simulink model "model_23b"  (R2023b)
settings: Solver=ode45  StartTime=TSPAN(1)  StopTime=TSPAN(2)  MaxStep=MaxStep  RelTol=RelTol  AbsTol=AbsTol
values from neighbouring files (symbols this model uses):
  dim_xp = numel(xp_0)    [init.m]
  JSPAN = [0 30*TSPAN(2)]    [init.m]
  parameters = struct()    [init.m]
  TSPAN = [0 600]    [init.m]
  xc_0 = [chi_0;theta_0]    [init.m]
  xp_0 = [p_0;q_0;v_0;o_0]    [init.m]
libraries: HyEQ_Library x2
settings Model: Creator=score  LastModifiedBy=zxz
settings DataIOCC: SaveFormat=Array  ReturnWorkspaceOutputs=off

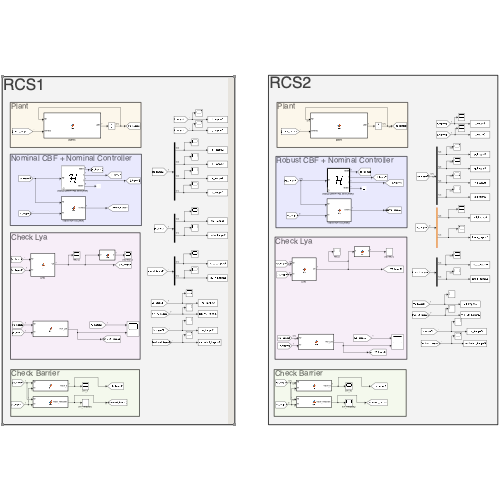
[thumbnail: Simulink's stored preview of the top-level diagram]
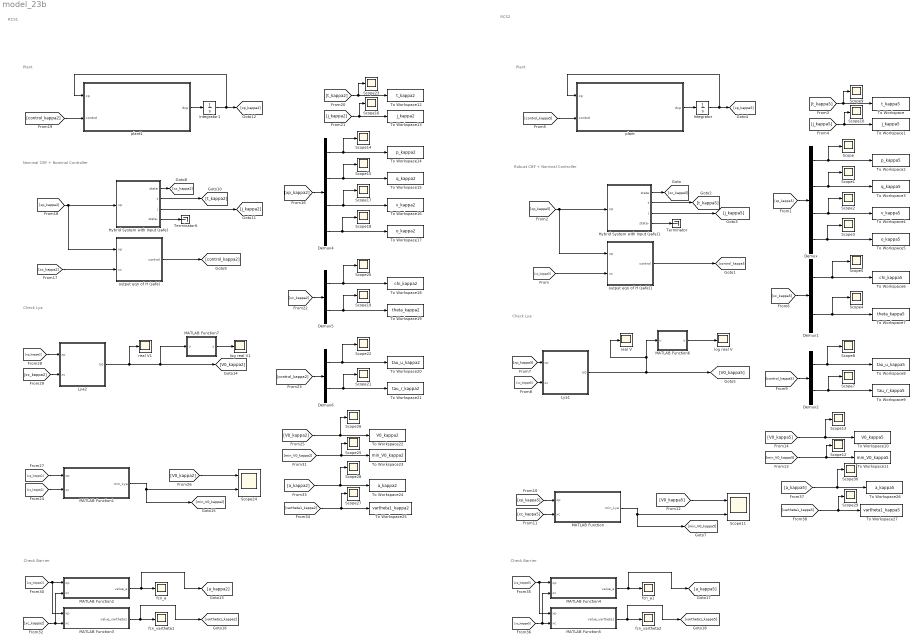
== system model_23b ==
  note: RCS2
  note: RCS1
  note: Check Barrier
  note: Check Lya
  note: Plant
  note: Robust CBF + Nominal Controller
  note: Plant
  note: Nominal CBF + Nominal Controller
  note: Check Lya
  note: Check Barrier
  Demux : Demux  Outputs=[2;2;2;1]
  Demux1 : Demux  Outputs=[2;1]
  Demux2 : Demux  Outputs=[1;1]
  Demux4 : Demux  Outputs=[2;2;2;1]
  Demux5 : Demux  Outputs=[2;1]
  Demux6 : Demux  Outputs=[1;1]
  Hybrid System with Input (safe) : Subsystem  LoadFcn=set_param(gcb,'LinkStatus','none')  mask(Hybrid System with Inputs){x0=xc_0, input_dim=dim_xp, parameters=parameters, T=TSPAN(2), J=JSPAN(2), rule=Flow}
      mask prompts: x0 "Initial Condition (column vector)"; input_dim "Input Dimension (positive integer)"; T "Flow Horizon (nonnegative real)"; J "Jump Horizon (nonnegative integer)"; rule "Flow/Jump Priorty Rule"
      mask help:
      | To modify (f, g, C, D) for this block, "Look inside" the block mask by either clicking the down arrow in the lower-left corner or selecting "Mask" > "Look Under Mask" from the context menu.
      |
      | For instructions how to use this block, see the
      mask init:
      | state_dim = numel(x0);
      settings: CopyFcn=|
      | set_param(gcb,'LinkStatus','none'),
      | set_param(gcs, 'MaxStep', 'MaxStep', 'RelTol', 'RelTol','StopTime', 'T')
      mask Help:
      | To modify (f, g, C, D) for this block, "Look inside" the block mask by either clicking the down arrow in the lower-left corner or selecting "Mask" > "Look Under Mask" from the context menu.
      | 
      | The value given in the 'parameters' field is passed as the last input argument for f, g, C, and D. Any MATLAB object can be used, but we recommend using a struct. For example, in the initialization script, a parameters struct can be defined as followed.
      |   parameters = struct();
      |   parameters.A = eye(2);
      |   parameters.B = [1; 0];
      | 
      | The output "x-" is the state output delayed by one integration step. Use this output to break algebraic loops.
      mask TypeOptions x0: Integrator System/x0
      mask TypeOptions T: Integrator System/T
      mask TypeOptions J: Integrator System/J
      mask TypeOptions rule: Jump | Flow | Random
      mask DialogControl Control2 Prompt: Introduction to the HyEQ Simulink-based Library
      mask DialogControl Control2 Callback: hybrid.internal.openHelp('Help_SimulinkLibrary')
      mask DialogControl Container3 Prompt: System Configuration
      mask DialogControl Container2 Prompt: Solver Options
      mask Display:
      | image('Hcal.jpg')
      | port_label('output', 1, 'state')
      | port_label('output', 2, 't')
      | port_label('output', 3, 'j')
      | port_label('output', 4, 'state^-','texmode', 'on')
      | port_label('input', 1, 'xp')
  Hybrid System with Input (safe)1 : Subsystem  LoadFcn=set_param(gcb,'LinkStatus','none')  mask(Hybrid System with Inputs){x0=xc_0, input_dim=dim_xp, parameters=parameters, T=TSPAN(2), J=JSPAN(2), rule=Flow}
      mask prompts: x0 "Initial Condition (column vector)"; input_dim "Input Dimension (positive integer)"; T "Flow Horizon (nonnegative real)"; J "Jump Horizon (nonnegative integer)"; rule "Flow/Jump Priorty Rule"
      mask help:
      | To modify (f, g, C, D) for this block, "Look inside" the block mask by either clicking the down arrow in the lower-left corner or selecting "Mask" > "Look Under Mask" from the context menu.
      |
      | For instructions how to use this block, see the
      mask init:
      | state_dim = numel(x0);
      settings: CopyFcn=|
      | set_param(gcb,'LinkStatus','none'),
      | set_param(gcs, 'MaxStep', 'MaxStep', 'RelTol', 'RelTol','StopTime', 'T')
      mask Help:
      | To modify (f, g, C, D) for this block, "Look inside" the block mask by either clicking the down arrow in the lower-left corner or selecting "Mask" > "Look Under Mask" from the context menu.
      | 
      | The value given in the 'parameters' field is passed as the last input argument for f, g, C, and D. Any MATLAB object can be used, but we recommend using a struct. For example, in the initialization script, a parameters struct can be defined as followed.
      |   parameters = struct();
      |   parameters.A = eye(2);
      |   parameters.B = [1; 0];
      | 
      | The output "x-" is the state output delayed by one integration step. Use this output to break algebraic loops.
      mask TypeOptions x0: Integrator System/x0
      mask TypeOptions T: Integrator System/T
      mask TypeOptions J: Integrator System/J
      mask TypeOptions rule: Jump | Flow | Random
      mask DialogControl Control2 Prompt: Introduction to the HyEQ Simulink-based Library
      mask DialogControl Control2 Callback: hybrid.internal.openHelp('Help_SimulinkLibrary')
      mask DialogControl Container3 Prompt: System Configuration
      mask DialogControl Container2 Prompt: Solver Options
      mask Display:
      | image('Hcal.jpg')
      | port_label('output', 1, 'state')
      | port_label('output', 2, 't')
      | port_label('output', 3, 'j')
      | port_label('output', 4, 'state^-','texmode', 'on')
      | port_label('input', 1, 'xp')
  Integrator : Integrator  InitialCondition=xp_0
  Integrator1 : Integrator  InitialCondition=xp_0
  Lya1 : MATLAB Function  TreatAsAtomicUnit=on
  Lya2 : MATLAB Function  TreatAsAtomicUnit=on
  MATLAB Function : MATLAB Function  TreatAsAtomicUnit=on
  MATLAB Function1 : MATLAB Function  TreatAsAtomicUnit=on
  MATLAB Function2 : MATLAB Function  TreatAsAtomicUnit=on
  MATLAB Function3 : MATLAB Function  TreatAsAtomicUnit=on
  MATLAB Function4 : MATLAB Function  TreatAsAtomicUnit=on
  MATLAB Function5 : MATLAB Function  TreatAsAtomicUnit=on
  MATLAB Function6 : MATLAB Function  TreatAsAtomicUnit=on
  MATLAB Function7 : MATLAB Function  TreatAsAtomicUnit=on
  Scope{,1..5,7..10,12..23,25..30} (28 alike) : Scope
  Scope11 : Scope  NumInputPorts=2
  Scope24 : Scope  NumInputPorts=2
  Terminator : Terminator
  Terminator6 : Terminator
  To Workspace : ToWorkspace  VariableName=t_kappa5  SaveFormat=Structure  SampleTime=-1
      settings: Save2DSignal=2-D array (concatenate along first dimension)
  To Workspace1 : ToWorkspace  VariableName=j_kappa5  SaveFormat=Structure  SampleTime=-1
      settings: Save2DSignal=2-D array (concatenate along first dimension)
  To Workspace10 : ToWorkspace  VariableName=V0_kappa5  SaveFormat=Structure  SampleTime=-1
      settings: Save2DSignal=2-D array (concatenate along first dimension)
  To Workspace11 : ToWorkspace  VariableName=min_V0_kappa5  SaveFormat=Structure  SampleTime=-1
      settings: Save2DSignal=2-D array (concatenate along first dimension)
  To Workspace12 : ToWorkspace  VariableName=t_kappa2  SaveFormat=Structure  SampleTime=-1
      settings: Save2DSignal=2-D array (concatenate along first dimension)
  To Workspace13 : ToWorkspace  VariableName=j_kappa2  SaveFormat=Structure  SampleTime=-1
      settings: Save2DSignal=2-D array (concatenate along first dimension)
  To Workspace14 : ToWorkspace  VariableName=p_kappa2  SaveFormat=Structure  SampleTime=-1
      settings: Save2DSignal=2-D array (concatenate along first dimension)
  To Workspace15 : ToWorkspace  VariableName=q_kappa2  SaveFormat=Structure  SampleTime=-1
      settings: Save2DSignal=2-D array (concatenate along first dimension)
  To Workspace16 : ToWorkspace  VariableName=v_kappa2  SaveFormat=Structure  SampleTime=-1
      settings: Save2DSignal=2-D array (concatenate along first dimension)
  To Workspace17 : ToWorkspace  VariableName=o_kappa2  SaveFormat=Structure  SampleTime=-1
      settings: Save2DSignal=2-D array (concatenate along first dimension)
  To Workspace18 : ToWorkspace  VariableName=chi_kappa2  SaveFormat=Structure  SampleTime=-1
      settings: Save2DSignal=2-D array (concatenate along first dimension)
  To Workspace19 : ToWorkspace  VariableName=theta_kappa2  SaveFormat=Structure  SampleTime=-1
      settings: Save2DSignal=2-D array (concatenate along first dimension)
  To Workspace2 : ToWorkspace  VariableName=p_kappa5  SaveFormat=Structure  SampleTime=-1
      settings: Save2DSignal=2-D array (concatenate along first dimension)
  To Workspace20 : ToWorkspace  VariableName=tau_u_kappa2  SaveFormat=Structure  SampleTime=-1
      settings: Save2DSignal=2-D array (concatenate along first dimension)
  To Workspace21 : ToWorkspace  VariableName=tau_r_kappa2  SaveFormat=Structure  SampleTime=-1
      settings: Save2DSignal=2-D array (concatenate along first dimension)
  To Workspace22 : ToWorkspace  VariableName=V0_kappa2  SaveFormat=Structure  SampleTime=-1
      settings: Save2DSignal=2-D array (concatenate along first dimension)
  To Workspace23 : ToWorkspace  VariableName=min_V0_kappa2  SaveFormat=Structure  SampleTime=-1
      settings: Save2DSignal=2-D array (concatenate along first dimension)
  To Workspace24 : ToWorkspace  VariableName=a_kappa2  SaveFormat=Structure  SampleTime=-1
      settings: Save2DSignal=2-D array (concatenate along first dimension)
  To Workspace25 : ToWorkspace  VariableName=vartheta1_kappa2  SaveFormat=Structure  SampleTime=-1
      settings: Save2DSignal=2-D array (concatenate along first dimension)
  To Workspace26 : ToWorkspace  VariableName=a_kappa5  SaveFormat=Structure  SampleTime=-1
      settings: Save2DSignal=2-D array (concatenate along first dimension)
  To Workspace27 : ToWorkspace  VariableName=vartheta1_kappa5  SaveFormat=Structure  SampleTime=-1
      settings: Save2DSignal=2-D array (concatenate along first dimension)
  To Workspace3 : ToWorkspace  VariableName=q_kappa5  SaveFormat=Structure  SampleTime=-1
      settings: Save2DSignal=2-D array (concatenate along first dimension)
  To Workspace4 : ToWorkspace  VariableName=v_kappa5  SaveFormat=Structure  SampleTime=-1
      settings: Save2DSignal=2-D array (concatenate along first dimension)
  To Workspace5 : ToWorkspace  VariableName=o_kappa5  SaveFormat=Structure  SampleTime=-1
      settings: Save2DSignal=2-D array (concatenate along first dimension)
  To Workspace6 : ToWorkspace  VariableName=chi_kappa5  SaveFormat=Structure  SampleTime=-1
      settings: Save2DSignal=2-D array (concatenate along first dimension)
  To Workspace7 : ToWorkspace  VariableName=theta_kappa5  SaveFormat=Structure  SampleTime=-1
      settings: Save2DSignal=2-D array (concatenate along first dimension)
  To Workspace8 : ToWorkspace  VariableName=tau_u_kappa5  SaveFormat=Structure  SampleTime=-1
      settings: Save2DSignal=2-D array (concatenate along first dimension)
  To Workspace9 : ToWorkspace  VariableName=tau_r_kappa5  SaveFormat=Structure  SampleTime=-1
      settings: Save2DSignal=2-D array (concatenate along first dimension)
  fcn_a : Scope
  fcn_a1 : Scope
  fcn_vartheta1 : Scope
  fcn_vartheta2 : Scope
  log real V : Scope
  log real V1 : Scope
  output eqn of H (safe) : MATLAB Function  TreatAsAtomicUnit=on
  output eqn of H (safe)1 : MATLAB Function  TreatAsAtomicUnit=on
  plant : MATLAB Function  TreatAsAtomicUnit=on
  plant1 : MATLAB Function  TreatAsAtomicUnit=on
  real V : Scope
  real V1 : Scope
  wires:
  Hybrid System with Input (safe)1/4(state-) -> Terminator/1
  Hybrid System with Input (safe)1/2(t) -> [t_kappa5]
  Hybrid System with Input (safe)1/3(j) -> [j_kappa5]
  Hybrid System with Input (safe)1/1(state) -> [xc_kappa5]
  [xp_kappa5] -> output eqn of H (safe)1/1(xp), Hybrid System with Input (safe)1/1(xp)
  [xc_kappa5] -> output eqn of H (safe)1/2(xc)
  output eqn of H (safe)1/1(control) -> [control_kappa5]
  [t_kappa5] -> Scope9/1, To Workspace/1
  [j_kappa5] -> Scope10/1, To Workspace1/1
  plant/1(dxp) -> Integrator/1
  [control_kappa5] -> plant/2(control)
  Integrator/1 -> plant/1(xp), [xp_kappa5]
  [xp_kappa5] -> Demux/1
  [xc_kappa5] -> Demux1/1
  Demux/1 -> Scope/1, To Workspace2/1
  Demux/2 -> Scope1/1, To Workspace3/1
  Demux/3 -> Scope2/1, To Workspace4/1
  Demux/4 -> Scope3/1, To Workspace5/1
  Demux1/2 -> To Workspace7/1, Scope4/1
  Demux1/1 -> Scope5/1, To Workspace6/1
  [xp_kappa5] -> Lya1/1(xp)
  [xc_kappa5] -> Lya1/2(xc)
  Lya1/1(V0) -> [V0_kappa5], MATLAB Function6/1(u), real V/1
  [control_kappa5] -> Demux2/1
  Demux2/2 -> Scope7/1, To Workspace9/1
  Demux2/1 -> To Workspace8/1, Scope8/1
  [xp_kappa5] -> MATLAB Function/1(xp)
  [xc_kappa5] -> MATLAB Function/2(xc)
  MATLAB Function/1(min_Lya) -> Scope11/2, [min_V0_kappa5]
  [V0_kappa5] -> Scope11/1
  [V0_kappa5] -> Scope13/1, To Workspace10/1
  [min_V0_kappa5] -> Scope12/1, To Workspace11/1
  output eqn of H (safe)/1(control) -> [control_kappa2]
  Hybrid System with Input (safe)/3(j) -> [j_kappa2]
  [xc_kappa2] -> output eqn of H (safe)/2(xc)
  [control_kappa2] -> plant1/2(control)
  Hybrid System with Input (safe)/2(t) -> [t_kappa2]
  Hybrid System with Input (safe)/1(state) -> [xc_kappa2]
  [xp_kappa2] -> output eqn of H (safe)/1(xp), Hybrid System with Input (safe)/1(xp)
  plant1/1(dxp) -> Integrator1/1
  Hybrid System with Input (safe)/4(state-) -> Terminator6/1
  Integrator1/1 -> plant1/1(xp), [xp_kappa2]
  Demux5/2 -> Scope19/1, To Workspace19/1
  [xc_kappa2] -> Demux5/1
  [t_kappa2] -> Scope23/1, To Workspace12/1
  [control_kappa2] -> Demux6/1
  Demux5/1 -> Scope20/1, To Workspace18/1
  Demux4/1 -> Scope14/1, To Workspace14/1
  [xp_kappa2] -> Demux4/1
  Demux4/2 -> Scope15/1, To Workspace15/1
  Demux4/3 -> Scope17/1, To Workspace16/1
  Demux4/4 -> Scope18/1, To Workspace17/1
  [j_kappa2] -> Scope16/1, To Workspace13/1
  Demux6/1 -> To Workspace20/1, Scope22/1
  Demux6/2 -> Scope21/1, To Workspace21/1
  MATLAB Function1/1(min_Lya) -> Scope24/2, [min_V0_kappa2]
  [xp_kappa2] -> MATLAB Function1/1(xp)
  [xc_kappa2] -> Lya2/2(xc)
  [xp_kappa2] -> Lya2/1(xp)
  [V0_kappa2] -> Scope24/1
  [xc_kappa2] -> MATLAB Function1/2(xc)
  [min_V0_kappa2] -> Scope25/1, To Workspace23/1
  [V0_kappa2] -> Scope26/1, To Workspace22/1
  [xp_kappa2] -> MATLAB Function3/1(xp), MATLAB Function2/1(xp)
  [xc_kappa2] -> MATLAB Function2/2(xc), MATLAB Function3/2(xc)
  MATLAB Function3/1(value_vartheta1) -> [vartheta1_kappa2], fcn_vartheta1/1
  MATLAB Function2/1(value_a) -> [a_kappa2], fcn_a/1
  [vartheta1_kappa2] -> Scope27/1, To Workspace25/1
  [a_kappa2] -> Scope28/1, To Workspace24/1
  [xp_kappa5] -> MATLAB Function5/1(xp), MATLAB Function4/1(xp)
  MATLAB Function4/1(value_a) -> [a_kappa5], fcn_a1/1
  [xc_kappa5] -> MATLAB Function4/2(xc), MATLAB Function5/2(xc)
  MATLAB Function5/1(value_vartheta1) -> [vartheta1_kappa5], fcn_vartheta2/1
  [vartheta1_kappa5] -> Scope29/1, To Workspace27/1
  [a_kappa5] -> Scope30/1, To Workspace26/1
  MATLAB Function6/1(y) -> log real V/1
  Lya2/1(V0) -> MATLAB Function7/1(u), [V0_kappa2], real V1/1
  MATLAB Function7/1(y) -> log real V1/1

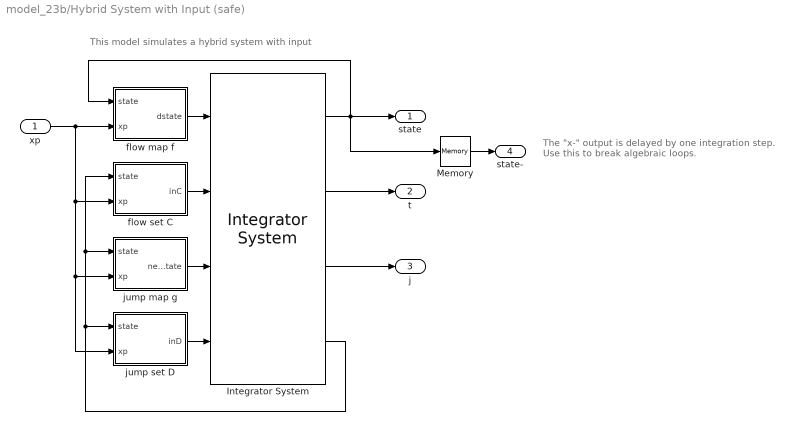
== system model_23b/Hybrid System with Input (safe) ==
  note: This model simulates a hybrid system with input
  note: The "x-" output is delayed by one integration step. Use this to break algebraic loops.
  xp : Inport  PortDimensions=input_dim
  Integrator System : HyEQ_Library/Other/Integrator System  Priority=2  T=T  J=J  x0=x0  rule=rule
      link override ICx: Value=xc_0
      link override ICx0: Value=[0; 0; xc_0(:)]
      settings: SourceProductName=Hybrid Equations Toolbox
  Memory : Memory  InitialCondition=x0
  flow map f : MATLAB Function  TreatAsAtomicUnit=on
  flow set C : MATLAB Function  TreatAsAtomicUnit=on
  jump map g : MATLAB Function  TreatAsAtomicUnit=on
  jump set D : MATLAB Function  TreatAsAtomicUnit=on
  state : Outport  PortDimensions=state_dim
  t : Outport  Port=2  PortDimensions=1
  j : Outport  Port=3  PortDimensions=1
  state- : Outport  Port=4  PortDimensions=state_dim
  wires:
  Memory/1 -> state-/1
  jump map g/1(nextstate) -> Integrator System/3
  jump set D/1(inD) -> Integrator System/4
  xp/1 -> jump set D/2(xp), jump map g/2(xp), flow set C/2(xp), flow map f/2(xp)
  Integrator System/3 -> j/1
  Integrator System/2 -> t/1
  flow set C/1(inC) -> Integrator System/2
  Integrator System/1 -> state/1, flow map f/1(state), Memory/1
  Integrator System/4 -> jump set D/1(state), jump map g/1(state), flow set C/1(state)
  flow map f/1(dstate) -> Integrator System/1

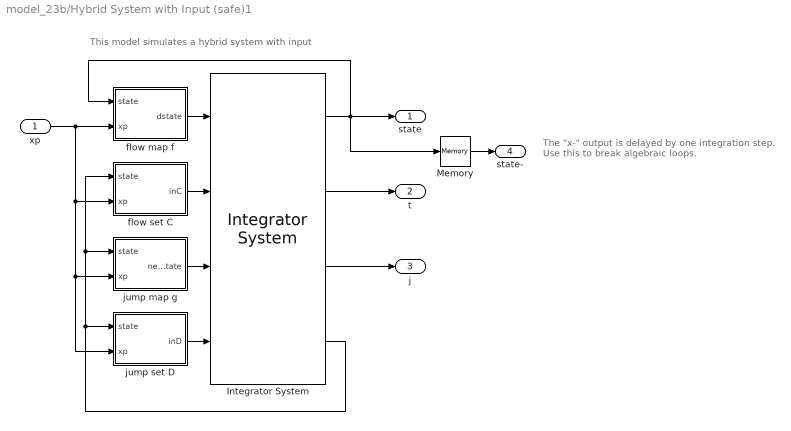
== system model_23b/Hybrid System with Input (safe)1 ==
  note: This model simulates a hybrid system with input
  note: The "x-" output is delayed by one integration step. Use this to break algebraic loops.
  xp : Inport  PortDimensions=input_dim
  Integrator System : HyEQ_Library/Other/Integrator System  Priority=2  T=T  J=J  x0=x0  rule=rule
      link override ICx: Value=xc_0
      link override ICx0: Value=[0; 0; xc_0(:)]
      settings: SourceProductName=Hybrid Equations Toolbox
  Memory : Memory  InitialCondition=x0
  flow map f : MATLAB Function  TreatAsAtomicUnit=on
  flow set C : MATLAB Function  TreatAsAtomicUnit=on
  jump map g : MATLAB Function  TreatAsAtomicUnit=on
  jump set D : MATLAB Function  TreatAsAtomicUnit=on
  state : Outport  PortDimensions=state_dim
  t : Outport  Port=2  PortDimensions=1
  j : Outport  Port=3  PortDimensions=1
  state- : Outport  Port=4  PortDimensions=state_dim
  wires:
  Memory/1 -> state-/1
  jump map g/1(nextstate) -> Integrator System/3
  jump set D/1(inD) -> Integrator System/4
  xp/1 -> jump set D/2(xp), jump map g/2(xp), flow set C/2(xp), flow map f/2(xp)
  Integrator System/3 -> j/1
  Integrator System/2 -> t/1
  flow set C/1(inC) -> Integrator System/2
  Integrator System/1 -> state/1, flow map f/1(state), Memory/1
  Integrator System/4 -> jump set D/1(state), jump map g/1(state), flow set C/1(state)
  flow map f/1(dstate) -> Integrator System/1

== matlab function model_23b/plant ==
  data: xp input; dxp output; control input; parameters parameter
function dxp = fcn(xp,control,parameters)

dxp=f_p(xp,control,parameters);

end

== matlab function model_23b/Hybrid System with Input (safe)/jump set D ==
  data: state input size=state_dim; xp input size=input_dim; inD output size=1; parameters parameter
function inD = D(state, xp, parameters)
   [~,inD]=fcn_decide(state,xp,parameters);
end

== matlab function model_23b/output eqn of H (safe) ==
  data: xp input; control output; xc input; parameters parameter
function control = fcn(xp,xc,parameters)

x0=[xp;xc];

control=kappa_2(x0,parameters);

end

== matlab function model_23b/plant1 ==
  data: xp input; dxp output; control input; parameters parameter
function dxp = fcn(xp,control,parameters)

dxp=f_p(xp,control,parameters);

end

== matlab function model_23b/MATLAB Function2 ==
  data: xp input; value_a output; xc input; parameters parameter
function value_a = fcn(xp,xc,parameters)

x0=[xp;xc];

value_a=a(x0,parameters);

end

== matlab function model_23b/MATLAB Function3 ==
  data: xp input; value_vartheta1 output; xc input; parameters parameter
function value_vartheta1 = fcn(xp,xc,parameters)

x0=[xp;xc];

value_vartheta1=vartheta1(x0,parameters);

end

== matlab function model_23b/MATLAB Function4 ==
  data: xp input; value_a output; xc input; parameters parameter
function value_a = fcn(xp,xc,parameters)

x0=[xp;xc(1:3)];

value_a=a(x0,parameters);

end

== matlab function model_23b/MATLAB Function5 ==
  data: xp input; value_vartheta1 output; xc input; parameters parameter
function value_vartheta1 = fcn(xp,xc,parameters)

x0=[xp;xc(1:3)];

value_vartheta1=vartheta1(x0,parameters);

end

== matlab function model_23b/MATLAB Function6 ==
  data: u input; y output
function y = fcn(u)

y = log(u+eps);

== matlab function model_23b/Lya2 ==
  data: xp input; V0 output; xc input; parameters parameter
function V0 = fcn(xp,xc,parameters)

x0=[xp;xc];

V0=fcn_V0(x0,parameters);

end

== matlab function model_23b/MATLAB Function7 ==
  data: u input; y output
function y = fcn(u)

y = log(u+eps);

== matlab function model_23b/MATLAB Function1 ==
  data: xp input; xc input; min_Lya output; parameters parameter
function min_Lya = fcn(xp,xc,parameters)

%%%
chi=xc(1:2);
% theta=state(3);

%%%
x0_0=[xp;chi;0];%theta=0
x0_1=[xp;chi;1];%theta=1
V0_0=fcn_V0(x0_0,parameters);%theta=0
V0_1=fcn_V0(x0_1,parameters);%theta=1

min_Lya=min(V0_0,V0_1);

end

== matlab function model_23b/Lya1 ==
  data: xp input; V0 output; xc input; parameters parameter
function V0 = fcn(xp,xc,parameters)

x0=[xp;xc];

V0=fcn_V0(x0,parameters);

end

== matlab function model_23b/output eqn of H (safe)1 ==
  data: xp input; control output; xc input; parameters parameter
function control = fcn(xp,xc,parameters)

x0=[xp;xc];

control=kappa_5(x0,parameters);

end

== matlab function model_23b/Hybrid System with Input (safe)1/flow map f ==
  data: state input size=state_dim; xp input size=input_dim; dstate output size=state_dim; parameters parameter
function dstate = f(state, xp, parameters)

dstate=f_flow(state, xp, parameters);

end

== matlab function model_23b/Hybrid System with Input (safe)1/flow set C ==
  data: state input size=state_dim; xp input size=input_dim; inC output size=1; parameters parameter
function inC = C(state, xp, parameters)
   [inC,~]=fcn_decide(state,xp,parameters);
end

== matlab function model_23b/Hybrid System with Input (safe)1/jump map g ==
  data: state input size=state_dim; xp input size=input_dim; nextstate output size=state_dim; parameters parameter
function nextstate = g(state, xp, parameters)

nextstate=f_jump(state, xp, parameters);

end

== matlab function model_23b/Hybrid System with Input (safe)1/jump set D ==
  data: state input size=state_dim; xp input size=input_dim; inD output size=1; parameters parameter
function inD = D(state, xp, parameters)
   [~,inD]=fcn_decide(state,xp,parameters);
end

== matlab function model_23b/MATLAB Function ==
  data: xp input; xc input; min_Lya output; parameters parameter
function min_Lya = fcn(xp,xc,parameters)

%%%
chi=xc(1:2);
% theta=state(3);

%%%
x0_0=[xp;chi;0];%theta=0
x0_1=[xp;chi;1];%theta=1
V0_0=fcn_V0(x0_0,parameters);%theta=0
V0_1=fcn_V0(x0_1,parameters);%theta=1

min_Lya=min(V0_0,V0_1);

end

== matlab function model_23b/Hybrid System with Input (safe)/flow map f ==
  data: state input size=state_dim; xp input size=input_dim; dstate output size=state_dim; parameters parameter
function dstate = f(state, xp, parameters)

dstate=f_flow(state, xp, parameters);

end

== matlab function model_23b/Hybrid System with Input (safe)/flow set C ==
  data: state input size=state_dim; xp input size=input_dim; inC output size=1; parameters parameter
function inC = C(state, xp, parameters)
   [inC,~]=fcn_decide(state,xp,parameters);
end

== matlab function model_23b/Hybrid System with Input (safe)/jump map g ==
  data: state input size=state_dim; xp input size=input_dim; nextstate output size=state_dim; parameters parameter
function nextstate = g(state, xp, parameters)

nextstate=f_jump(state, xp, parameters);

end
